simulink model "milestone1"  (R2026a)
settings: Solver=FixedStepAuto  StopTime=100  EnableMultiTasking=on
libraries: arduinolib x2, simulink x1
settings Model: SimulationMode=external  SILPILModeSetting=veronly  ExtModeTrigDuration=2  Creator=ejarr  LastModifiedBy=ejarr
settings HardwareCC: ProdBitPerInt=16.0  ProdBitPerPointer=16.0  ProdBitPerSizeT=16.0  ProdBitPerPtrDiffT=16.0  ProdWordSize=8.0  ProdHWDeviceType=Atmel->AVR  UseEmbeddedCoderFeatures=off  UseSimulinkCoderFeatures=off
settings RTWCC: SystemTargetFile=ert.tlc  HardwareBoard=Arduino Mega 2560  TLCOptions=-aInlineSetEventsForThisBaseRateFcn=TLC_FALSE -aSuppressMultiTaskScheduler=TLC_FALSE -aRateBasedStepFcn=1  Toolchain=Arduino AVR  BuildConfiguration=Faster Runs  Description=Embedded Coder
settings CodeAppCC: MangleLength=10.0
settings ERTTargetCC: ExtModeTransport=3.0  ExtModeAutomaticAllocSize=off  ExtModeStaticAllocSize=2048.0  SupportContinuousTime=on  SupportNonInlinedSFcns=on  SupportVariableSizeSignals=on

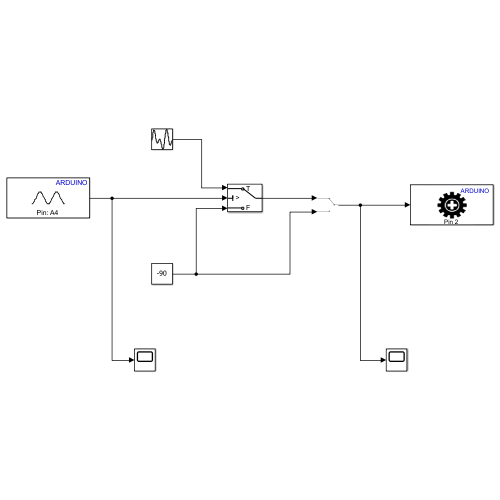
[thumbnail: Simulink's stored preview of the top-level diagram]
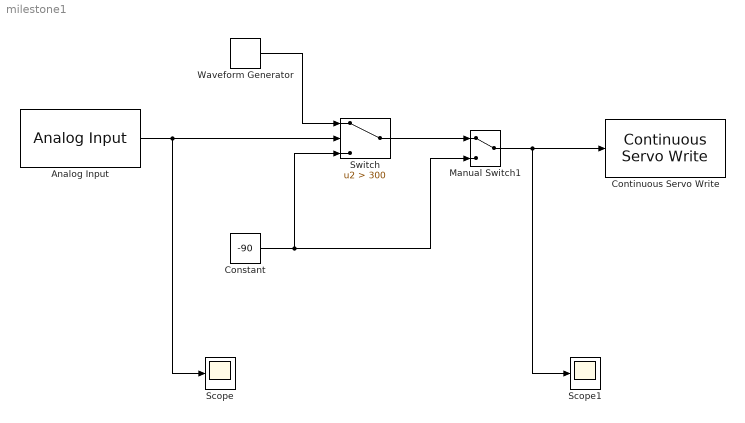
== system milestone1 ==
  Analog Input : arduinolib/Analog Input  pinNumber=4  ReadResultsOnly=off  ConversionTriggerSource=Software  ExternalTriggerType=uint32( 0 )  OutputDataType=uint16  EnableConversionCompleteNotify=off  EnableOuputStatus=off  SampleTime=-1  blockPlatform=arduino
      settings: LibrarySourceBlock=gizmoLibrary/Arduino Utilities/Analog Input
  Constant : Constant  Value=-90
  Continuous Servo Write : arduinolib/Continuous Servo Write  pinNumber=2  ServoIndex=0  blockPlatform=ARDUINO
  Manual Switch1 : ManualSwitch
  Scope : Scope
      settings: ActiveDisplayYMinimum=-1223.1373780694746  ActiveDisplayYMaximum=1489.6765391133652
  Scope1 : Scope
      settings: ActiveDisplayYMinimum=-62.434985333353609  ActiveDisplayYMaximum=52.884436226698234
  Switch : Switch  Criteria=u2 > Threshold  Threshold=300  SaturateOnIntegerOverflow=off  InputSameDT=off
  Waveform Generator : simulink/Sources/Waveform Generator  OutMin=[]  OutMax=[]  OutDataTypeStr=double  SelectedSignal=1  Signals=sin(90, 3, 1)  BlockNames=MultiportSwitch_47339956ce674cc  SampleTime=0.1
  wires:
  Waveform Generator/1 -> Switch/1
  Analog Input/1 -> Scope/1, Switch/2
  Switch/1 -> Manual Switch1/1
  Manual Switch1/1 -> Scope1/1, Continuous Servo Write/1
  Constant/1 -> Switch/3, Manual Switch1/2
